simulink model "self_balancing_robot_pid_rebuilt"  (R2026b)
settings: Solver=VariableStepAuto  StopTime=15
values from neighbouring files (symbols this model uses):
  a = M + m    (= 0.72)    [robot_params.m]
  b = m*l    (= 0.0726)    [robot_params.m]
  c = I + m*l^2    (= 0.029958)    [robot_params.m]
  disturbance_end = 4.1    [compare_pid_lqr.m]    (also in compare_v3.m = distEnd_list(i); version3_analysis.m = 5.1)
  disturbance_mag = 0.5    [compare_pid_lqr.m]    (also in compare_v3.m = distMag_list(i); version3_analysis.m = 0)
  disturbance_start = 4    [compare_pid_lqr.m]    (also in compare_v3.m = distStart_list(i); version3_analysis.m)
  g = 9.81    [robot_params.m]
  initial_tilt = deg2rad(5)    [compare_pid_lqr.m]
  l = 0.33    [robot_params.m]
  m = 0.22    [robot_params.m]
  q = a*c - b^2    (= 0.016299)    [robot_params.m]
settings Model: Creator=legne  LastModifiedBy=legne

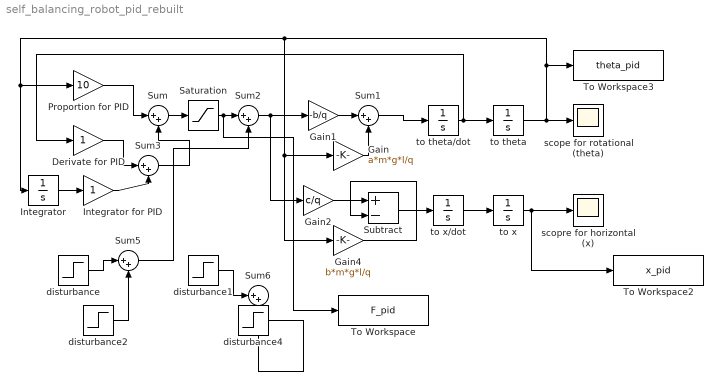
== system self_balancing_robot_pid_rebuilt ==
  Derivate for PID : Gain
  Gain : Gain  Gain=a*m*g*l/q
  Gain1 : Gain  Gain=-b/q
  Gain2 : Gain  Gain=c/q
  Gain4 : Gain  Gain=b*m*g*l/q
  Integrator : Integrator
  Integrator for PID : Gain
  Proportion for PID : Gain  Gain=10
  Saturation : Saturate  UpperLimit=2  LowerLimit=-2
  Subtract : Sum  Inputs=+-
  Sum{,1..3,5..6} (6 alike) : Sum  Inputs=|++
  To Workspace : ToWorkspace  VariableName=F_pid  SaveFormat=Timeseries  SampleTime=-1
  To Workspace2 : ToWorkspace  VariableName=x_pid  SaveFormat=Timeseries  SampleTime=-1
  To Workspace3 : ToWorkspace  VariableName=theta_pid  SaveFormat=Timeseries  SampleTime=-1
  disturbance : Step  Time=disturbance_start  FinalValue=disturbance_mag  SampleTime=0
  disturbance1 : Step  Time=7  FinalValue=0.5  SampleTime=0
  disturbance2 : Step  Time=disturbance_end  FinalValue=-disturbance_mag  SampleTime=0
  disturbance4 : Step  Time=7.1  FinalValue=-0.5  SampleTime=0
  scope for rotational (theta) : Scope
      settings: ActiveDisplayYMinimum=-0.28069761812399019  ActiveDisplayYMaximum=0.48695238474875696
  scopre for horizontal (x) : Scope
      settings: ActiveDisplayYMinimum=-8.2019282658323842  ActiveDisplayYMaximum=2.0078504367294778
  to theta : Integrator  InitialCondition=initial_tilt
  to theta/dot : Integrator
  to x : Integrator
  to x/dot : Integrator
  wires:
  Gain/1 -> Sum1/2
  to theta/dot/1 -> Derivate for PID/1, to theta/1
  to theta/1 -> To Workspace3/1, Integrator/1, Proportion for PID/1, Gain/1, Gain4/1, scope for rotational (theta)/1
  Gain1/1 -> Sum1/1
  Sum1/1 -> to theta/dot/1
  Gain2/1 -> Subtract/1
  Subtract/1 -> to x/dot/1
  to x/dot/1 -> to x/1
  to x/1 -> scopre for horizontal (x)/1, To Workspace2/1
  Gain4/1 -> Subtract/2
  Proportion for PID/1 -> Sum/1
  Sum/1 -> Saturation/1
  Saturation/1 -> To Workspace/1, Sum2/1
  Sum2/1 -> Gain1/1, Gain2/1
  Integrator/1 -> Integrator for PID/1
  Sum3/1 -> Sum/2
  Derivate for PID/1 -> Sum3/1
  Integrator for PID/1 -> Sum3/2
  disturbance2/1 -> Sum5/2
  disturbance/1 -> Sum5/1
  disturbance1/1 -> Sum6/1
  disturbance4/1 -> Sum6/2
  Sum5/1 -> Sum2/2
